simulink model "furuta_rl_training"  (R2026b)
settings: Solver=FixedStepDiscrete  StopTime=5  FixedStep=controlPeriod
model workspace (MAT data in the model file):
  agentKind : string (value not decoded)
  controlPeriod = 0.01
  controllerMode = 1
  furutaAgent : rl.agent.rlPPOAgent (value not decoded)
  furutaToolboxMpc : object (value not decoded)
  initialState = [0; 0.174532925199; 0; 0]
  integrationStep = 0.002
  lmpcF = [-2830.68997815 -2386.43056313 -2007.92623528 -1685.61022299 -1411.30389107 -1178.01505811 -979.765570681 -811.443882151 -668.67900017 -547.732694122 -445.407303829 -358.966875555 ... (80 elements, 20x4)]
  lmpcH = [71196.7632757 60515.4631775 51389.63963 43592.1776843 36929.7000861 31236.7872342 26371.8858267 22213.8049684 18658.7129743 15617.560407 13013.8653496 10781.8057824 ... (400 elements, 20x20)]
  lqrGain = [-0.560244322113 -7.30813603654 -0.304541725168 -0.68699829167]
  maxTorque = 0.03
  pidGains = [8.3479 0.5085 0.5811 0.3312 0.0475]
  plantCoefficients = [0.00019818 0.00016078 0.00016134 0.00013805 0.016934 0.0001 1e-05 0]
  poleGain = [-1.34079378819 -10.2715412157 -0.553426126336 -0.956316780761]
  rlRewardLevel = 2
  rmd : object (value not decoded)
  rmdCommandDelaySamples = 1
  rmdCurrentTimeConstant = 0
  scenarioStimulus = [0 0.0075 0.0175 0.0275 0.0375 0.0475 0.0575 0.0675 0.0775 0.0875 0.0975 0.1075 ... (2004 elements, 501x4)]
  usePolicyCallback = 0
  useRmd = 1
symbols that are objects in the model workspace (value not decoded): rmd
undefined symbols (not defined in the file or in its folder): sgn
libraries: mpclib x1, rllib x1
(part 2 of 2)

== system furuta_rl_training/05 Furuta plant/RK4 Furuta plant/Substep 3/k3 ==
  x : Inport
  tau : Inport  Port=2
  Arm acceleration : Fcn  Expr=(u(3)*u(4)-u(2)*u(5))/(u(1)*u(3)-(u(2)*u(2)))
  Arm rate : Fcn  Expr=u(3)
  D11 : Fcn  Expr=u(6)+u(7)*(sin(u(2))*sin(u(2)))
  D12 : Fcn  Expr=u(9)*cos(u(2))
  D22 : Fcn  Expr=u(8)
  Mass matrix and RHS : Mux  Inputs=5
  Pend acceleration : Fcn  Expr=(u(1)*u(5)-u(2)*u(4))/(u(1)*u(3)-(u(2)*u(2)))
  Pend rate : Fcn  Expr=u(4)
  Physical parameters : Constant  Value=plantCoefficients
  State derivative : Mux
  State torque parameters : Mux  Inputs=3
  Torque RHS arm : Fcn  Expr=u(5)-2*u(7)*sin(u(2))*cos(u(2))*u(3)*u(4)+u(9)*sin(u(2))*(u(4)*u(4))-u(11)*u(3)-u(13)*sgn(u(3))
  Torque RHS pend : Fcn  Expr=u(7)*sin(u(2))*cos(u(2))*(u(3)*u(3))-u(12)*u(4)+u(10)*sin(u(2))
  xdot : Outport
  wires:
  x/1 -> State torque parameters/1
  tau/1 -> State torque parameters/2
  Physical parameters/1 -> State torque parameters/3
  State torque parameters/1 -> D11/1, D12/1, D22/1, Torque RHS arm/1, Torque RHS pend/1, Arm rate/1, Pend rate/1
  D11/1 -> Mass matrix and RHS/1
  D12/1 -> Mass matrix and RHS/2
  D22/1 -> Mass matrix and RHS/3
  Torque RHS arm/1 -> Mass matrix and RHS/4
  Torque RHS pend/1 -> Mass matrix and RHS/5
  Arm rate/1 -> State derivative/1
  Pend rate/1 -> State derivative/2
  Mass matrix and RHS/1 -> Arm acceleration/1, Pend acceleration/1
  Arm acceleration/1 -> State derivative/3
  Pend acceleration/1 -> State derivative/4
  State derivative/1 -> xdot/1

== system furuta_rl_training/05 Furuta plant/RK4 Furuta plant/Substep 3/k4 ==
  x : Inport
  tau : Inport  Port=2
  Arm acceleration : Fcn  Expr=(u(3)*u(4)-u(2)*u(5))/(u(1)*u(3)-(u(2)*u(2)))
  Arm rate : Fcn  Expr=u(3)
  D11 : Fcn  Expr=u(6)+u(7)*(sin(u(2))*sin(u(2)))
  D12 : Fcn  Expr=u(9)*cos(u(2))
  D22 : Fcn  Expr=u(8)
  Mass matrix and RHS : Mux  Inputs=5
  Pend acceleration : Fcn  Expr=(u(1)*u(5)-u(2)*u(4))/(u(1)*u(3)-(u(2)*u(2)))
  Pend rate : Fcn  Expr=u(4)
  Physical parameters : Constant  Value=plantCoefficients
  State derivative : Mux
  State torque parameters : Mux  Inputs=3
  Torque RHS arm : Fcn  Expr=u(5)-2*u(7)*sin(u(2))*cos(u(2))*u(3)*u(4)+u(9)*sin(u(2))*(u(4)*u(4))-u(11)*u(3)-u(13)*sgn(u(3))
  Torque RHS pend : Fcn  Expr=u(7)*sin(u(2))*cos(u(2))*(u(3)*u(3))-u(12)*u(4)+u(10)*sin(u(2))
  xdot : Outport
  wires:
  x/1 -> State torque parameters/1
  tau/1 -> State torque parameters/2
  Physical parameters/1 -> State torque parameters/3
  State torque parameters/1 -> D11/1, D12/1, D22/1, Torque RHS arm/1, Torque RHS pend/1, Arm rate/1, Pend rate/1
  D11/1 -> Mass matrix and RHS/1
  D12/1 -> Mass matrix and RHS/2
  D22/1 -> Mass matrix and RHS/3
  Torque RHS arm/1 -> Mass matrix and RHS/4
  Torque RHS pend/1 -> Mass matrix and RHS/5
  Arm rate/1 -> State derivative/1
  Pend rate/1 -> State derivative/2
  Mass matrix and RHS/1 -> Arm acceleration/1, Pend acceleration/1
  Arm acceleration/1 -> State derivative/3
  Pend acceleration/1 -> State derivative/4
  State derivative/1 -> xdot/1

== system furuta_rl_training/05 Furuta plant/RK4 Furuta plant/Substep 4/k1 ==
  x : Inport
  tau : Inport  Port=2
  Arm acceleration : Fcn  Expr=(u(3)*u(4)-u(2)*u(5))/(u(1)*u(3)-(u(2)*u(2)))
  Arm rate : Fcn  Expr=u(3)
  D11 : Fcn  Expr=u(6)+u(7)*(sin(u(2))*sin(u(2)))
  D12 : Fcn  Expr=u(9)*cos(u(2))
  D22 : Fcn  Expr=u(8)
  Mass matrix and RHS : Mux  Inputs=5
  Pend acceleration : Fcn  Expr=(u(1)*u(5)-u(2)*u(4))/(u(1)*u(3)-(u(2)*u(2)))
  Pend rate : Fcn  Expr=u(4)
  Physical parameters : Constant  Value=plantCoefficients
  State derivative : Mux
  State torque parameters : Mux  Inputs=3
  Torque RHS arm : Fcn  Expr=u(5)-2*u(7)*sin(u(2))*cos(u(2))*u(3)*u(4)+u(9)*sin(u(2))*(u(4)*u(4))-u(11)*u(3)-u(13)*sgn(u(3))
  Torque RHS pend : Fcn  Expr=u(7)*sin(u(2))*cos(u(2))*(u(3)*u(3))-u(12)*u(4)+u(10)*sin(u(2))
  xdot : Outport
  wires:
  State derivative/1 -> xdot/1
  Pend acceleration/1 -> State derivative/4
  Arm acceleration/1 -> State derivative/3
  Mass matrix and RHS/1 -> Pend acceleration/1, Arm acceleration/1
  Pend rate/1 -> State derivative/2
  Arm rate/1 -> State derivative/1
  Torque RHS pend/1 -> Mass matrix and RHS/5
  Torque RHS arm/1 -> Mass matrix and RHS/4
  D22/1 -> Mass matrix and RHS/3
  D12/1 -> Mass matrix and RHS/2
  D11/1 -> Mass matrix and RHS/1
  State torque parameters/1 -> Pend rate/1, Arm rate/1, Torque RHS pend/1, Torque RHS arm/1, D22/1, D12/1, D11/1
  Physical parameters/1 -> State torque parameters/3
  tau/1 -> State torque parameters/2
  x/1 -> State torque parameters/1

== system furuta_rl_training/05 Furuta plant/RK4 Furuta plant/Substep 4/k2 ==
  x : Inport
  tau : Inport  Port=2
  Arm acceleration : Fcn  Expr=(u(3)*u(4)-u(2)*u(5))/(u(1)*u(3)-(u(2)*u(2)))
  Arm rate : Fcn  Expr=u(3)
  D11 : Fcn  Expr=u(6)+u(7)*(sin(u(2))*sin(u(2)))
  D12 : Fcn  Expr=u(9)*cos(u(2))
  D22 : Fcn  Expr=u(8)
  Mass matrix and RHS : Mux  Inputs=5
  Pend acceleration : Fcn  Expr=(u(1)*u(5)-u(2)*u(4))/(u(1)*u(3)-(u(2)*u(2)))
  Pend rate : Fcn  Expr=u(4)
  Physical parameters : Constant  Value=plantCoefficients
  State derivative : Mux
  State torque parameters : Mux  Inputs=3
  Torque RHS arm : Fcn  Expr=u(5)-2*u(7)*sin(u(2))*cos(u(2))*u(3)*u(4)+u(9)*sin(u(2))*(u(4)*u(4))-u(11)*u(3)-u(13)*sgn(u(3))
  Torque RHS pend : Fcn  Expr=u(7)*sin(u(2))*cos(u(2))*(u(3)*u(3))-u(12)*u(4)+u(10)*sin(u(2))
  xdot : Outport
  wires:
  x/1 -> State torque parameters/1
  tau/1 -> State torque parameters/2
  Physical parameters/1 -> State torque parameters/3
  State torque parameters/1 -> D11/1, D12/1, D22/1, Torque RHS arm/1, Torque RHS pend/1, Arm rate/1, Pend rate/1
  D11/1 -> Mass matrix and RHS/1
  D12/1 -> Mass matrix and RHS/2
  D22/1 -> Mass matrix and RHS/3
  Torque RHS arm/1 -> Mass matrix and RHS/4
  Torque RHS pend/1 -> Mass matrix and RHS/5
  Arm rate/1 -> State derivative/1
  Pend rate/1 -> State derivative/2
  Mass matrix and RHS/1 -> Arm acceleration/1, Pend acceleration/1
  Arm acceleration/1 -> State derivative/3
  Pend acceleration/1 -> State derivative/4
  State derivative/1 -> xdot/1

== system furuta_rl_training/05 Furuta plant/RK4 Furuta plant/Substep 4/k3 ==
  x : Inport
  tau : Inport  Port=2
  Arm acceleration : Fcn  Expr=(u(3)*u(4)-u(2)*u(5))/(u(1)*u(3)-(u(2)*u(2)))
  Arm rate : Fcn  Expr=u(3)
  D11 : Fcn  Expr=u(6)+u(7)*(sin(u(2))*sin(u(2)))
  D12 : Fcn  Expr=u(9)*cos(u(2))
  D22 : Fcn  Expr=u(8)
  Mass matrix and RHS : Mux  Inputs=5
  Pend acceleration : Fcn  Expr=(u(1)*u(5)-u(2)*u(4))/(u(1)*u(3)-(u(2)*u(2)))
  Pend rate : Fcn  Expr=u(4)
  Physical parameters : Constant  Value=plantCoefficients
  State derivative : Mux
  State torque parameters : Mux  Inputs=3
  Torque RHS arm : Fcn  Expr=u(5)-2*u(7)*sin(u(2))*cos(u(2))*u(3)*u(4)+u(9)*sin(u(2))*(u(4)*u(4))-u(11)*u(3)-u(13)*sgn(u(3))
  Torque RHS pend : Fcn  Expr=u(7)*sin(u(2))*cos(u(2))*(u(3)*u(3))-u(12)*u(4)+u(10)*sin(u(2))
  xdot : Outport
  wires:
  x/1 -> State torque parameters/1
  tau/1 -> State torque parameters/2
  Physical parameters/1 -> State torque parameters/3
  State torque parameters/1 -> D11/1, D12/1, D22/1, Torque RHS arm/1, Torque RHS pend/1, Arm rate/1, Pend rate/1
  D11/1 -> Mass matrix and RHS/1
  D12/1 -> Mass matrix and RHS/2
  D22/1 -> Mass matrix and RHS/3
  Torque RHS arm/1 -> Mass matrix and RHS/4
  Torque RHS pend/1 -> Mass matrix and RHS/5
  Arm rate/1 -> State derivative/1
  Pend rate/1 -> State derivative/2
  Mass matrix and RHS/1 -> Arm acceleration/1, Pend acceleration/1
  Arm acceleration/1 -> State derivative/3
  Pend acceleration/1 -> State derivative/4
  State derivative/1 -> xdot/1

== system furuta_rl_training/05 Furuta plant/RK4 Furuta plant/Substep 4/k4 ==
  x : Inport
  tau : Inport  Port=2
  Arm acceleration : Fcn  Expr=(u(3)*u(4)-u(2)*u(5))/(u(1)*u(3)-(u(2)*u(2)))
  Arm rate : Fcn  Expr=u(3)
  D11 : Fcn  Expr=u(6)+u(7)*(sin(u(2))*sin(u(2)))
  D12 : Fcn  Expr=u(9)*cos(u(2))
  D22 : Fcn  Expr=u(8)
  Mass matrix and RHS : Mux  Inputs=5
  Pend acceleration : Fcn  Expr=(u(1)*u(5)-u(2)*u(4))/(u(1)*u(3)-(u(2)*u(2)))
  Pend rate : Fcn  Expr=u(4)
  Physical parameters : Constant  Value=plantCoefficients
  State derivative : Mux
  State torque parameters : Mux  Inputs=3
  Torque RHS arm : Fcn  Expr=u(5)-2*u(7)*sin(u(2))*cos(u(2))*u(3)*u(4)+u(9)*sin(u(2))*(u(4)*u(4))-u(11)*u(3)-u(13)*sgn(u(3))
  Torque RHS pend : Fcn  Expr=u(7)*sin(u(2))*cos(u(2))*(u(3)*u(3))-u(12)*u(4)+u(10)*sin(u(2))
  xdot : Outport
  wires:
  x/1 -> State torque parameters/1
  tau/1 -> State torque parameters/2
  Physical parameters/1 -> State torque parameters/3
  State torque parameters/1 -> D11/1, D12/1, D22/1, Torque RHS arm/1, Torque RHS pend/1, Arm rate/1, Pend rate/1
  D11/1 -> Mass matrix and RHS/1
  D12/1 -> Mass matrix and RHS/2
  D22/1 -> Mass matrix and RHS/3
  Torque RHS arm/1 -> Mass matrix and RHS/4
  Torque RHS pend/1 -> Mass matrix and RHS/5
  Arm rate/1 -> State derivative/1
  Pend rate/1 -> State derivative/2
  Mass matrix and RHS/1 -> Arm acceleration/1, Pend acceleration/1
  Arm acceleration/1 -> State derivative/3
  Pend acceleration/1 -> State derivative/4
  State derivative/1 -> xdot/1

== system furuta_rl_training/05 Furuta plant/RK4 Furuta plant/Substep 5/k1 ==
  x : Inport
  tau : Inport  Port=2
  Arm acceleration : Fcn  Expr=(u(3)*u(4)-u(2)*u(5))/(u(1)*u(3)-(u(2)*u(2)))
  Arm rate : Fcn  Expr=u(3)
  D11 : Fcn  Expr=u(6)+u(7)*(sin(u(2))*sin(u(2)))
  D12 : Fcn  Expr=u(9)*cos(u(2))
  D22 : Fcn  Expr=u(8)
  Mass matrix and RHS : Mux  Inputs=5
  Pend acceleration : Fcn  Expr=(u(1)*u(5)-u(2)*u(4))/(u(1)*u(3)-(u(2)*u(2)))
  Pend rate : Fcn  Expr=u(4)
  Physical parameters : Constant  Value=plantCoefficients
  State derivative : Mux
  State torque parameters : Mux  Inputs=3
  Torque RHS arm : Fcn  Expr=u(5)-2*u(7)*sin(u(2))*cos(u(2))*u(3)*u(4)+u(9)*sin(u(2))*(u(4)*u(4))-u(11)*u(3)-u(13)*sgn(u(3))
  Torque RHS pend : Fcn  Expr=u(7)*sin(u(2))*cos(u(2))*(u(3)*u(3))-u(12)*u(4)+u(10)*sin(u(2))
  xdot : Outport
  wires:
  State derivative/1 -> xdot/1
  Pend acceleration/1 -> State derivative/4
  Arm acceleration/1 -> State derivative/3
  Mass matrix and RHS/1 -> Pend acceleration/1, Arm acceleration/1
  Pend rate/1 -> State derivative/2
  Arm rate/1 -> State derivative/1
  Torque RHS pend/1 -> Mass matrix and RHS/5
  Torque RHS arm/1 -> Mass matrix and RHS/4
  D22/1 -> Mass matrix and RHS/3
  D12/1 -> Mass matrix and RHS/2
  D11/1 -> Mass matrix and RHS/1
  State torque parameters/1 -> Pend rate/1, Arm rate/1, Torque RHS pend/1, Torque RHS arm/1, D22/1, D12/1, D11/1
  Physical parameters/1 -> State torque parameters/3
  tau/1 -> State torque parameters/2
  x/1 -> State torque parameters/1

== system furuta_rl_training/05 Furuta plant/RK4 Furuta plant/Substep 5/k2 ==
  x : Inport
  tau : Inport  Port=2
  Arm acceleration : Fcn  Expr=(u(3)*u(4)-u(2)*u(5))/(u(1)*u(3)-(u(2)*u(2)))
  Arm rate : Fcn  Expr=u(3)
  D11 : Fcn  Expr=u(6)+u(7)*(sin(u(2))*sin(u(2)))
  D12 : Fcn  Expr=u(9)*cos(u(2))
  D22 : Fcn  Expr=u(8)
  Mass matrix and RHS : Mux  Inputs=5
  Pend acceleration : Fcn  Expr=(u(1)*u(5)-u(2)*u(4))/(u(1)*u(3)-(u(2)*u(2)))
  Pend rate : Fcn  Expr=u(4)
  Physical parameters : Constant  Value=plantCoefficients
  State derivative : Mux
  State torque parameters : Mux  Inputs=3
  Torque RHS arm : Fcn  Expr=u(5)-2*u(7)*sin(u(2))*cos(u(2))*u(3)*u(4)+u(9)*sin(u(2))*(u(4)*u(4))-u(11)*u(3)-u(13)*sgn(u(3))
  Torque RHS pend : Fcn  Expr=u(7)*sin(u(2))*cos(u(2))*(u(3)*u(3))-u(12)*u(4)+u(10)*sin(u(2))
  xdot : Outport
  wires:
  x/1 -> State torque parameters/1
  tau/1 -> State torque parameters/2
  Physical parameters/1 -> State torque parameters/3
  State torque parameters/1 -> D11/1, D12/1, D22/1, Torque RHS arm/1, Torque RHS pend/1, Arm rate/1, Pend rate/1
  D11/1 -> Mass matrix and RHS/1
  D12/1 -> Mass matrix and RHS/2
  D22/1 -> Mass matrix and RHS/3
  Torque RHS arm/1 -> Mass matrix and RHS/4
  Torque RHS pend/1 -> Mass matrix and RHS/5
  Arm rate/1 -> State derivative/1
  Pend rate/1 -> State derivative/2
  Mass matrix and RHS/1 -> Arm acceleration/1, Pend acceleration/1
  Arm acceleration/1 -> State derivative/3
  Pend acceleration/1 -> State derivative/4
  State derivative/1 -> xdot/1

== system furuta_rl_training/05 Furuta plant/RK4 Furuta plant/Substep 5/k3 ==
  x : Inport
  tau : Inport  Port=2
  Arm acceleration : Fcn  Expr=(u(3)*u(4)-u(2)*u(5))/(u(1)*u(3)-(u(2)*u(2)))
  Arm rate : Fcn  Expr=u(3)
  D11 : Fcn  Expr=u(6)+u(7)*(sin(u(2))*sin(u(2)))
  D12 : Fcn  Expr=u(9)*cos(u(2))
  D22 : Fcn  Expr=u(8)
  Mass matrix and RHS : Mux  Inputs=5
  Pend acceleration : Fcn  Expr=(u(1)*u(5)-u(2)*u(4))/(u(1)*u(3)-(u(2)*u(2)))
  Pend rate : Fcn  Expr=u(4)
  Physical parameters : Constant  Value=plantCoefficients
  State derivative : Mux
  State torque parameters : Mux  Inputs=3
  Torque RHS arm : Fcn  Expr=u(5)-2*u(7)*sin(u(2))*cos(u(2))*u(3)*u(4)+u(9)*sin(u(2))*(u(4)*u(4))-u(11)*u(3)-u(13)*sgn(u(3))
  Torque RHS pend : Fcn  Expr=u(7)*sin(u(2))*cos(u(2))*(u(3)*u(3))-u(12)*u(4)+u(10)*sin(u(2))
  xdot : Outport
  wires:
  x/1 -> State torque parameters/1
  tau/1 -> State torque parameters/2
  Physical parameters/1 -> State torque parameters/3
  State torque parameters/1 -> D11/1, D12/1, D22/1, Torque RHS arm/1, Torque RHS pend/1, Arm rate/1, Pend rate/1
  D11/1 -> Mass matrix and RHS/1
  D12/1 -> Mass matrix and RHS/2
  D22/1 -> Mass matrix and RHS/3
  Torque RHS arm/1 -> Mass matrix and RHS/4
  Torque RHS pend/1 -> Mass matrix and RHS/5
  Arm rate/1 -> State derivative/1
  Pend rate/1 -> State derivative/2
  Mass matrix and RHS/1 -> Arm acceleration/1, Pend acceleration/1
  Arm acceleration/1 -> State derivative/3
  Pend acceleration/1 -> State derivative/4
  State derivative/1 -> xdot/1

== system furuta_rl_training/05 Furuta plant/RK4 Furuta plant/Substep 5/k4 ==
  x : Inport
  tau : Inport  Port=2
  Arm acceleration : Fcn  Expr=(u(3)*u(4)-u(2)*u(5))/(u(1)*u(3)-(u(2)*u(2)))
  Arm rate : Fcn  Expr=u(3)
  D11 : Fcn  Expr=u(6)+u(7)*(sin(u(2))*sin(u(2)))
  D12 : Fcn  Expr=u(9)*cos(u(2))
  D22 : Fcn  Expr=u(8)
  Mass matrix and RHS : Mux  Inputs=5
  Pend acceleration : Fcn  Expr=(u(1)*u(5)-u(2)*u(4))/(u(1)*u(3)-(u(2)*u(2)))
  Pend rate : Fcn  Expr=u(4)
  Physical parameters : Constant  Value=plantCoefficients
  State derivative : Mux
  State torque parameters : Mux  Inputs=3
  Torque RHS arm : Fcn  Expr=u(5)-2*u(7)*sin(u(2))*cos(u(2))*u(3)*u(4)+u(9)*sin(u(2))*(u(4)*u(4))-u(11)*u(3)-u(13)*sgn(u(3))
  Torque RHS pend : Fcn  Expr=u(7)*sin(u(2))*cos(u(2))*(u(3)*u(3))-u(12)*u(4)+u(10)*sin(u(2))
  xdot : Outport
  wires:
  x/1 -> State torque parameters/1
  tau/1 -> State torque parameters/2
  Physical parameters/1 -> State torque parameters/3
  State torque parameters/1 -> D11/1, D12/1, D22/1, Torque RHS arm/1, Torque RHS pend/1, Arm rate/1, Pend rate/1
  D11/1 -> Mass matrix and RHS/1
  D12/1 -> Mass matrix and RHS/2
  D22/1 -> Mass matrix and RHS/3
  Torque RHS arm/1 -> Mass matrix and RHS/4
  Torque RHS pend/1 -> Mass matrix and RHS/5
  Arm rate/1 -> State derivative/1
  Pend rate/1 -> State derivative/2
  Mass matrix and RHS/1 -> Arm acceleration/1, Pend acceleration/1
  Arm acceleration/1 -> State derivative/3
  Pend acceleration/1 -> State derivative/4
  State derivative/1 -> xdot/1

== matlab function furuta_rl_training/03 Controllers/PID with anti windup ==
  data: x input; u output; g input; dt input; mode input
function u = pid(x,g,dt,mode)
% 적분은 PID 모드에서만 갱신하고 입력 포화 방향에서는 누적하지 않는다.
persistent integral
if isempty(integral) || mode ~= 2
    integral = 0;
end
e = atan2(sin(x(2)),cos(x(2)));
base = g(1)*e+g(2)*x(4)+g(3)*x(1)+g(4)*x(3);
candidate = base+g(5)*(integral+dt*e);
if mode == 2 && (abs(candidate)<=1 || sign(candidate)~=sign(e))
    integral = integral+dt*e;
end
u = base+g(5)*integral;
end

== matlab function furuta_rl_training/03 Controllers/Policy callback ==
  data: x input; u output; t input; elapsed output; enabled input
function [u,elapsed] = control(x,t,enabled)
% 기본 LQR에서는 외부 MATLAB 함수를 실행하지 않는다.
coder.extrinsic('furuta_sl_context');
u = 0; elapsed = NaN;
if enabled >= 0.5
    [u,elapsed] = furuta_sl_context(x(:),t);
end
end

== matlab function furuta_rl_training/03 Controllers/RL observation reward termination ==
  data: x input; obs output; lastAction input; level input; mode input; reward output; done output
function [obs,reward,done] = observe(x,lastAction,level,mode)
% 상태는 현재 샘플, 보상에 쓰는 행동은 이전 샘플이다.
c = cos(x(2)); s = sin(x(2));
obs = [c;s;x(1);x(3);x(4)];
reward = c-0.01*lastAction^2;
if level == 2
    reward = reward-.001*x(4)^2-.00002*x(3)^2+double(abs(atan2(s,c))<.35);
end
done = mode == 5 && abs(x(1))>2*pi;
if done
    reward = -50;
end
end

== matlab function furuta_rl_training/03 Controllers/LMPC bounded QP ==
  data: x input; u output; mode input; H input; F input
function u = move(x,mode,H,F)
% 이전 해를 한 단계 이동해 재사용하고 모든 좌표를 [-1,1]로 제한한다.
persistent previous
if isempty(previous)
    previous = zeros(20,1);
end
u = 0;
if mode ~= 6
    previous(:) = 0;
    return
end
z = x(:);
z(2) = atan2(sin(z(2)),cos(z(2)));
f = F*z;
U = [previous(2:end); previous(end)];
gradient = H*U+f;
for it = 1:100
    change = 0;
    for j = 1:20
        next = min(1,max(-1,U(j)-gradient(j)/H(j,j)));
        step = next-U(j);
        U(j) = next;
        gradient = gradient+H(:,j)*step;
        change = max(change,abs(step));
    end
    if change<1e-7
        break
    end
end
previous = U;
u = U(1);
end
